simulink model "mpc1_1"  (R2016a)
settings: Solver=VariableStepAuto  StartTime=0.0  StopTime=10.0  MaxStep=10e-3  MinStep=10e-5  RelTol=1e-3
libraries: mpclib x1, cstblocks x1
settings Model: Creator=Mojtaba  LastModifiedBy=Mojtaba
settings SolverCC: InitialStep=10e-4
settings GRTTargetCC: GeneratePreprocessorConditionals=Use local settings

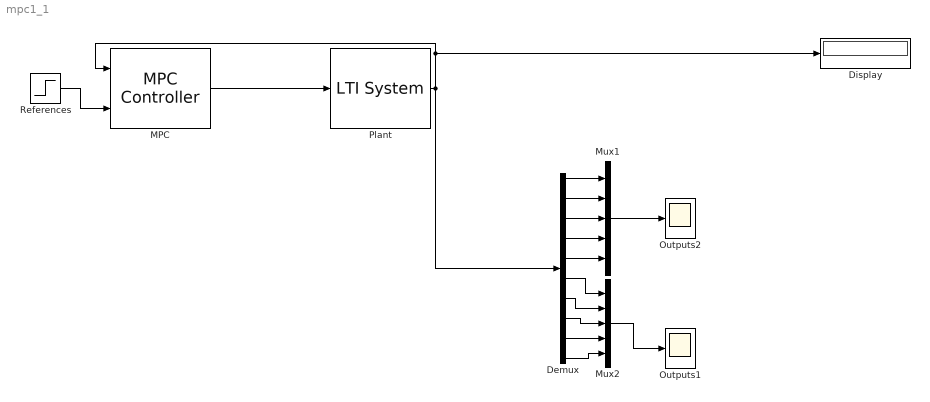
== system mpc1_1 ==
  Demux : Demux  Outputs=10
  Display : Display
  MPC : mpclib/MPC Controller  SCDEnableBlockLinearizationSpecification=on  mpcobj=mpc1_1_C  is_multiple=0  enable_value=0  return_u0=off  ref_from_ws=off  ref_signal_name=[]  ref_preview=off  md_from_ws=off  md_signal_name=[]  md_preview=off  from_project=off  project_file=MPCtask.mat  md_inport=off  mv_inport=off  cost_outport=off  return_sequence=off  return_qpstatus=off  return_state=off  state_inport=off  lims_inport=off  ywt_inport=off  is_designfromscratch=0  uwt_inport=off  duwt_inport=off  rhoeps_inport=off  uref_inport=off  n_ts=0.5  n_mv=5  n_md=0  n_ud=0  n_mo=10  n_uo=0  BlockDataType=double  SampleTimeInherited=off  switch_inport=off
  Mux1 : Mux  Inputs=5
  Mux2 : Mux  Inputs=5
  Outputs1 : Scope
  Outputs2 : Scope
  Plant : cstblocks/LTI System  sys=mpc1_1_G  IC=[]
  References : Step  Before=[0;0;0;0;0;0;0;0;0;0]  After=[1;1;1;1;1;1;1;1;1;1]
  wires:
  References/1 -> MPC/2
  MPC/1 -> Plant/1
  Plant/1 -> Display/1, MPC/1, Demux/1
  Demux/1 -> Mux1/1
  Demux/2 -> Mux1/2
  Demux/3 -> Mux1/3
  Demux/4 -> Mux1/4
  Demux/5 -> Mux1/5
  Demux/6 -> Mux2/1
  Demux/7 -> Mux2/2
  Demux/8 -> Mux2/3
  Demux/9 -> Mux2/4
  Demux/10 -> Mux2/5
  Mux1/1 -> Outputs2/1
  Mux2/1 -> Outputs1/1
